simulink model "ex7_uart"  (Simulink 7.6)
settings: Solver=FixedStepDiscrete  SolverMode=SingleTasking  StartTime=0.0  StopTime=10.0  FixedStep=0.001  RelTol=1e-3
libraries: dsPICdrivers x10
settings Model: Creator=Lior  LastModifiedBy=Lior  BufferReuse=off
settings OptimizationCC: BlockReduction=off  InlineParams=on  BufferReuse=off  OptimizeModelRefInitCode=on  LifeSpan=1
settings HardwareCC: ProdBitPerInt=16  ProdBitPerPointer=16  ProdEndianess=LittleEndian  ProdWordSize=16  ProdHWDeviceType=16-bit Generic
settings RTWCC: SystemTargetFile=dspic.tlc  GenCodeOnly=on  MakeCommand=make_CreateMPLAB  TemplateMakefile=dspic_pic30_gcc.tmf  PostCodeGenCommand=dsPIC_Compile()  Description=Embedded Target for Microchip dsPIC (real-time)  ProcessScript=dspic_make_rtw_hook
settings CodeAppCC: IgnoreCustomStorageClasses=off
settings STFCustomTargetCC: IncludeMdlTerminateFcn=off  CombineOutputUpdateFcns=on  SuppressErrorStatus=on  ERTCustomFileBanners=on  SupportContinuousTime=off  SupportNonInlinedSFcns=off  SystemTargetFile=dspic.tlc
settings ERTTargetCC: MultiwordLength=2048  ParMdlRefBuildCompliant=off  CompOptLevelCompliant=off  IncludeMdlTerminateFcn=off  SuppressErrorStatus=on  ERTFirstTimeCompliant=off  ModelStepFunctionPrototypeControlCompliant=off  CPPClassGenCompliant=off  ExtModeMexFile=ext_serial_win32_comm  InlinedParameterPlacement=NonHierarchical  ERTSrcFileBannerTemplate=dsPIC_code_template.cgt  ERTHdrFileBannerTemplate=dsPIC_code_template.cgt  ERTDataSrcFileTemplate=dsPIC_code_template.cgt  ERTDataHdrFileTemplate=dsPIC_code_template.cgt  ERTCustomFileTemplate=dsPIC_main.tlc  ConvertIfToSwitch=off
settings CustomProperty: DataType=string  Value=C:\PROGRA~1\MATLAB\R2010b\bin\win64\gmake

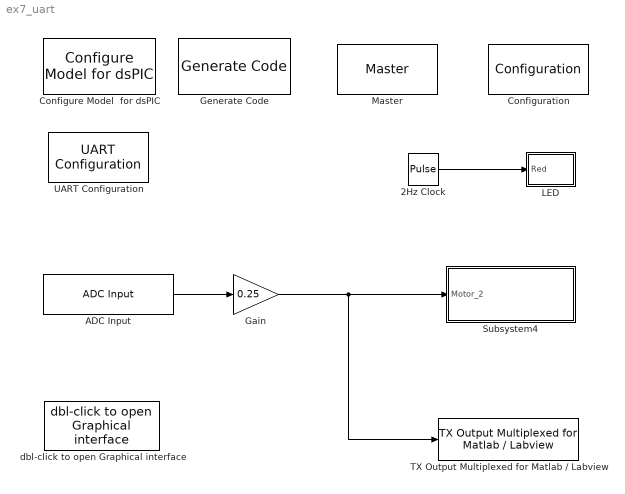
== system ex7_uart ==
  2Hz Clock : DiscretePulseGenerator  PulseType=Time based  Period=1  PulseWidth=50
  ADC Input : dsPICdrivers/Peripheral I//O/ADC Input  Tag=dsPIC_ADC  Priority=5  ADC_TYPE=10 bits  ADC_MODE=Continuous sampling & get last channel value  NbrSampleStep=1  VoltRefpopup="AVdd  -  AVss"  OutFormatBitspopup=0000 00dd dddd dddd : Integer  InterruptPriority=6  ANCHANNELS=[1]  MaxName=ANmax = 1023  Rin=1e2  ADCS=0  SAMC=1  Temperature=25  DMAChannel=4  SampleTime=-1  Status="OK  |  Tsmp=2.000e-007 |  T/Channel=2.600e-006 |  Tall=2.600e-006"  SSRC=auto convert
  Configuration : dsPICdrivers/Configuration  SystemSampleTime=-1  double64=off
  Configure Model  for dsPIC : dsPICdrivers/Simulink Configuration/Configure Model  for dsPIC
  Gain : Gain  Gain=0.25  OutDataTypeStr=uint8
  Generate Code : dsPICdrivers/Simulink Configuration/Generate Code
  LED : Subsystem
  Master : dsPICdrivers/Master  Tag=dsPIC_MASTER  Priority=1  TimeStepType=Timer1  picType=30f4011  fcy=2500000  Quartz_33f=5e6  PLLActive_33f=off  fcyDesired_33f=0  tmr1="[1  2499  0]"  tmr1Info="Time Step : 0.001  ;   Error : 0%  PR1=2499"  tmr2345="[0  0  0  0]"  tmr2345cfg=[-1 -1 -1 -1]  IOautoConf=on  typePort="[ 0   0   0   0   0   0   0   0   0   0   0   0   0   0   0   0  10   8   0   0   0   0   0   0   0   0   0   0   0   0   0   0   0   0   0   0   0   0   0   0   0   0   0   0   0   0   0   0   0   0   0   0   0   0   0   0   0   0   0   0   0   0   0   0   0   0   0   0   0   0   0   0   0   0   0   0   0   0   0   0   0   0  20  20   4   5   0   0   0   0   0   0   0   0   0   0   0   0   0   0   0   0   0   0   0   0   0   0   0   0   0   0 ]"  TRIS="[ 65535  65534  65535  65535  65535  65535  65535 ]"  ADPCFG=1  MasterBusyPort=None  MasterOverloadPort=None  FOSC=CSW_FSCM_OFF  ClockSwitchMonitor=Both disabled  TempProtection_33f=TEMP_ON  FPBOR=PBOR_OFF  PWRT=PWRT_OFF  MCLR=MCLR_EN  ICD=ICS_PGD1  JTAGEN=JTAGEN_OFF  PowerSave=off  OverrideFcy=off  NewFcy=1e6  PR2345="[65535  65535  65535  65535]"
  Subsystem4 : Subsystem  mask(Activate a motor via I2C){Motor_Add=6}
      mask prompts: Motor_Add "Motor Address"
      mask help: Please choose the motor that you want to activate
      mask StyleString: popup(1|2|3|4|5|6)
      mask Display: fprintf('Motor_%d \n\n Input speed [0-255]',Motor_Add)
  TX Output Multiplexed for Matlab / Labview : dsPICdrivers/Serial PORT/TX Output Multiplexed for Matlab // Labview  Tag=dsPIC_TX_Multiplexed  Priority=5  UART=2  CleverSpreadingChk=on  CleverSpreading=1  CHANNEL=[0]  CHANNELBLOCKED=[]  CHANNELBLOCKED_BITEWISE=0  Status=OK
  UART Configuration : dsPICdrivers/Serial PORT/UART Configuration  Tag=dsPIC_config_UART  Priority=2  UART=2  proposed_BAUD=9600  BAUD=9600  ALT_TX_RX=on  InterruptTxWhen=When Transmit Buffer is empty  TXInterruptPri=1  TxBufferSize=32  TXEN=on  InterruptRxWhen=When Receive Buffer is full (contain 4 characters)  RXInterruptPri=2  RxBufferSize=32  DoNotImplementRxInterrupt=off  DoNotImplementTxInterrupt=off  UxBRG=15  Info="UxBRG = 15   ||  Real Baud : 9766   ||  % error : 1.7253  ||  max 0.97656 Bytes / Step"  RealBaud=0  ERROR=1.7253  BYTES_STEP=0.97656
  dbl-click to open Graphical interface : dsPICdrivers/Serial PORT/dbl-click to open Graphical interface  Nothing=0
  wires:
  2Hz Clock/1 -> LED/1(Red)
  ADC Input/1 -> Gain/1
  Gain/1 -> Subsystem4/1(Motor_2), TX Output Multiplexed for Matlab / Labview/1

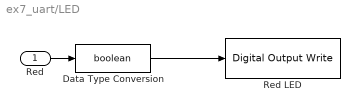
== system ex7_uart/LED ==
  Red : Inport
  Data Type Conversion : DataTypeConversion  OutDataTypeStr=boolean
  Red LED : dsPICdrivers/Digital I//O/Digital Output Write  Tag=dsPIC_Digital_Output  Priority=5  PORT=B  Pin=[0]  Simultaneous=off  OrderingInOutPopup=None
  wires:
  Data Type Conversion/1 -> Red LED/1
  Red/1 -> Data Type Conversion/1

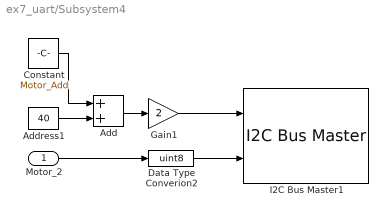
== system ex7_uart/Subsystem4 ==
  Motor_2 : Inport
  Add : Sum
  Address1 : Constant  Value=40  OutDataTypeStr=uint8
  Constant : Constant  Value=Motor_Add
  Data Type Converion2 : DataTypeConversion  OutDataTypeStr=uint8
  Gain1 : Gain  Gain=2  OutDataTypeStr=uint8
  I2C Bus Master1 : dsPICdrivers/BUS I2C/I2C Bus Master  Tag=dsPIC_I2C_Master  NumI2C=1  AltI2C=off  Sequence='S A W P'  InitializeOnceOnly=When I2C bus is enable (if Enable I2C is checked)  Enable=on  WaitAfterEnable=4  Disable=on  AdressNbrBits=7 bits  I2CBusFreq=153  SlewRate=off  SMBUSThreshold=off  OutputErrorFlag=off  SampleTime=0.01  OrderingInOutPopup=None  Info=Fscl = 16 KHz
  wires:
  Gain1/1 -> I2C Bus Master1/1
  Data Type Converion2/1 -> I2C Bus Master1/2
  Motor_2/1 -> Data Type Converion2/1
  Add/1 -> Gain1/1
  Constant/1 -> Add/1
  Address1/1 -> Add/2
